simulink model "TopOil_SunWind_50MVA"  (R2025a)
settings: Solver=ode4  StartTime=0.0  StopTime=Tstop  FixedStep=dt  RelTol=1e-3
values from neighbouring files (symbols this model uses):
  cA = p(3)    [step6_weather_extension.m]    (also in step7_results.mat = 22.4389421542; step7_sumgait_year.m = 22.4389421542; step8_simulink_sunwind.m = cases{i,2})
  dH0 = dHR * (K^2)^m    [step8_simulink_sunwind.m]    (also in step9_extend_thesis_model.m = p.dHR * (K^2)^p.m)
  dHR = 18    [step8_simulink_sunwind.m]
  dTOR = 49    [step8_simulink_sunwind.m]
  kw = p(4)    [step6_weather_extension.m]    (also in step7_results.mat = 0.0504; step7_sumgait_year.m = 0.0504; step8_simulink_sunwind.m = cases{i,3})
  m = 0.8    [Case2_inputs.m]    (also in step7_sumgait_year.m; step8_simulink_sunwind.m)
  n = 0.8    [Case2_inputs.m]    (also in step6_results.mat; step6_weather_extension.m; step7_sumgait_year.m; step8_simulink_sunwind.m)
  P_R = 136000    [step6_results.mat]    (also in step6_weather_extension.m; step7_sumgait_year.m = 162820; step8_simulink_sunwind.m = 162820)
  R = [0 1 2 3 4 5 6 7 8 9 10 11 ... (276 elements, 46x6)]    [SA1_sweep.mat]    (also in step10_SA1_continuous.m = zeros(nT, 6); step6_results.mat = 7.5; step6_weather_extension.m = 7.5; step7_sumgait_year.m = 5.04829123328)
  tauTO = 180*60    (= 10800)    [step8_simulink_sunwind.m]
  tauW = 6*60    (= 360)    [step8_simulink_sunwind.m]
  TO0 = TO(end)    [step10_SA1_continuous.m]    (also in step8_simulink_sunwind.m = Ta + dTOR * (U/(1 + kw*W))^n; step9_extend_thesis_model.m = Ta + p.dTOR * (U/(1 + p.kw*W))^p.n)
settings Model: Creator=Mahammad  LastModifiedBy=Mahammad

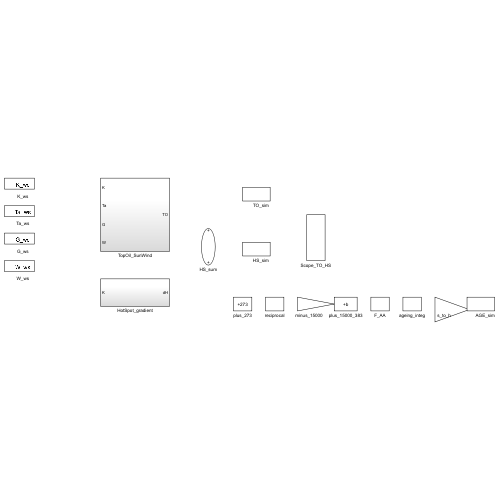
[thumbnail: Simulink's stored preview of the top-level diagram]
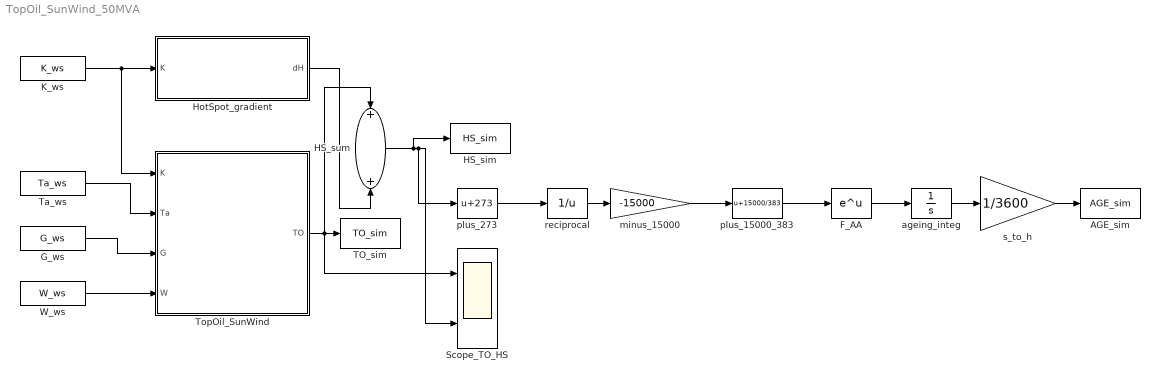
== system TopOil_SunWind_50MVA ==
  AGE_sim : ToWorkspace  VariableName=AGE_sim  SaveFormat=Structure With Time  SampleTime=-1
  F_AA : Math
  G_ws : FromWorkspace  VariableName=G_ws  OutputAfterFinalValue=Holding final value
  HS_sim : ToWorkspace  VariableName=HS_sim  SaveFormat=Structure With Time  SampleTime=-1
  HS_sum : Sum
  HotSpot_gradient : Subsystem
  K_ws : FromWorkspace  VariableName=K_ws  Interpolate=off  OutputAfterFinalValue=Holding final value
  Scope_TO_HS : Scope  NumInputPorts=2
  TO_sim : ToWorkspace  VariableName=TO_sim  SaveFormat=Structure With Time  SampleTime=-1
  Ta_ws : FromWorkspace  VariableName=Ta_ws  OutputAfterFinalValue=Holding final value
  TopOil_SunWind : Subsystem
  W_ws : FromWorkspace  VariableName=W_ws  OutputAfterFinalValue=Holding final value
  ageing_integ : Integrator
  minus_15000 : Gain  Gain=-15000
  plus_15000_383 : Bias  Bias=15000/383  SaturateOnIntegerOverflow=off
  plus_273 : Bias  Bias=273  SaturateOnIntegerOverflow=off
  reciprocal : Math  Operator=reciprocal
  s_to_h : Gain  Gain=1/3600
  wires:
  plus_273/1 -> reciprocal/1
  Ta_ws/1 -> TopOil_SunWind/2(Ta)
  HS_sum/1 -> Scope_TO_HS/2, plus_273/1, HS_sim/1
  plus_15000_383/1 -> F_AA/1
  W_ws/1 -> TopOil_SunWind/4(W)
  G_ws/1 -> TopOil_SunWind/3(G)
  reciprocal/1 -> minus_15000/1
  K_ws/1 -> TopOil_SunWind/1(K), HotSpot_gradient/1(K)
  HotSpot_gradient/1(dH) -> HS_sum/2
  TopOil_SunWind/1(TO) -> HS_sum/1, TO_sim/1, Scope_TO_HS/1
  minus_15000/1 -> plus_15000_383/1
  F_AA/1 -> ageing_integ/1
  ageing_integ/1 -> s_to_h/1
  s_to_h/1 -> AGE_sim/1

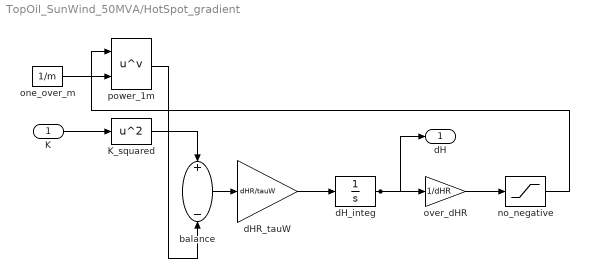
== system TopOil_SunWind_50MVA/HotSpot_gradient ==
  K : Inport
  K_squared : Math  Operator=square
  balance : Sum  Inputs=+-
  dHR_tauW : Gain  Gain=dHR/tauW
  dH_integ : Integrator  InitialCondition=dH0
  no_negative : Saturate  UpperLimit=inf  LowerLimit=0
  one_over_m : Constant  Value=1/m
  over_dHR : Gain  Gain=1/dHR
  power_1m : Math  Operator=pow
  dH : Outport
  wires:
  over_dHR/1 -> no_negative/1
  dH_integ/1 -> dH/1, over_dHR/1
  one_over_m/1 -> power_1m/2
  K/1 -> K_squared/1
  power_1m/1 -> balance/2
  dHR_tauW/1 -> dH_integ/1
  K_squared/1 -> balance/1
  balance/1 -> dHR_tauW/1
  no_negative/1 -> power_1m/1

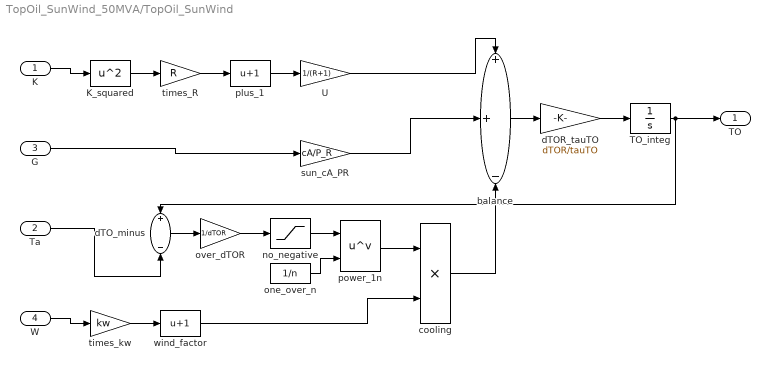
== system TopOil_SunWind_50MVA/TopOil_SunWind ==
  K : Inport
  Ta : Inport  Port=2
  G : Inport  Port=3
  W : Inport  Port=4
  K_squared : Math  Operator=square
  TO_integ : Integrator  InitialCondition=TO0
  U : Gain  Gain=1/(R+1)
  balance : Sum  Inputs=++-
  cooling : Product
  dTOR_tauTO : Gain  Gain=dTOR/tauTO
  dTO_minus : Sum  Inputs=+-
  no_negative : Saturate  UpperLimit=inf  LowerLimit=0
  one_over_n : Constant  Value=1/n
  over_dTOR : Gain  Gain=1/dTOR
  plus_1 : Bias  Bias=1  SaturateOnIntegerOverflow=off
  power_1n : Math  Operator=pow
  sun_cA_PR : Gain  Gain=cA/P_R
  times_R : Gain  Gain=R
  times_kw : Gain  Gain=kw
  wind_factor : Bias  Bias=1  SaturateOnIntegerOverflow=off
  TO : Outport
  wires:
  K/1 -> K_squared/1
  K_squared/1 -> times_R/1
  times_R/1 -> plus_1/1
  plus_1/1 -> U/1
  U/1 -> balance/1
  G/1 -> sun_cA_PR/1
  sun_cA_PR/1 -> balance/2
  W/1 -> times_kw/1
  times_kw/1 -> wind_factor/1
  TO_integ/1 -> dTO_minus/1, TO/1
  Ta/1 -> dTO_minus/2
  dTO_minus/1 -> over_dTOR/1
  over_dTOR/1 -> no_negative/1
  no_negative/1 -> power_1n/1
  one_over_n/1 -> power_1n/2
  power_1n/1 -> cooling/1
  wind_factor/1 -> cooling/2
  cooling/1 -> balance/3
  balance/1 -> dTOR_tauTO/1
  dTOR_tauTO/1 -> TO_integ/1
